simulink subsystem "Driving"  (R2024a)
settings: Solver=VariableStepAuto  StartTime=0.0  StopTime=10.0  RelTol=1e-3
settings Model: Creator=User  LastModifiedBy=User

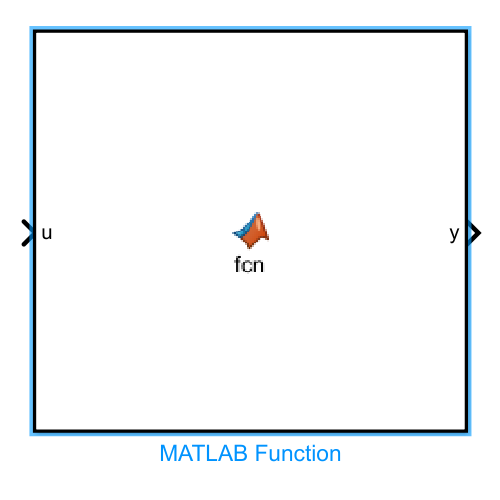
[thumbnail: Simulink's stored preview of the top-level diagram]
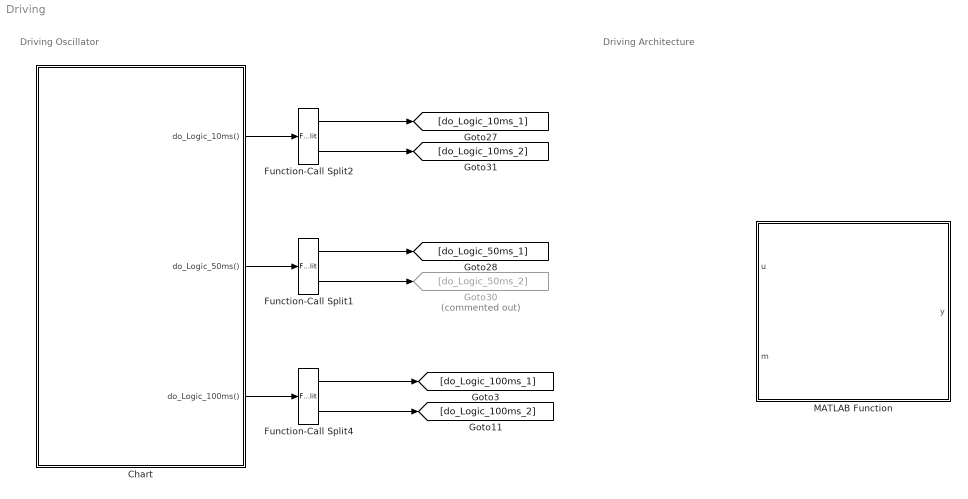
== system Driving ==
  note: Driving Oscillator
  note: Driving Architecture
  Chart : Stateflow chart  TreatAsAtomicUnit=on
  Function-Call Split1 : FunctionCallSplit  IconShape=distinctive  NumOutputPorts=2  OutputPortLayout=default
  Function-Call Split2 : FunctionCallSplit  IconShape=distinctive  NumOutputPorts=2  OutputPortLayout=default
  Function-Call Split4 : FunctionCallSplit  IconShape=distinctive  NumOutputPorts=2  OutputPortLayout=default
  Goto30 : Goto  Commented=on  GotoTag=do_Logic_50ms_2
  MATLAB Function : MATLAB Function  TreatAsAtomicUnit=on
  wires:
  Function-Call Split4/2 -> [do_Logic_100ms_2]
  Function-Call Split4/1 -> [do_Logic_100ms_1]
  Function-Call Split1/1 -> [do_Logic_50ms_1]
  Chart/3(do_Logic_100ms()) -> Function-Call Split4/1
  Function-Call Split2/2 -> [do_Logic_10ms_2]
  Function-Call Split1/2 -> Goto30/1
  Function-Call Split2/1 -> [do_Logic_10ms_1]
  Chart/2(do_Logic_50ms()) -> Function-Call Split1/1
  Chart/1(do_Logic_10ms()) -> Function-Call Split2/1

== matlab function Driving/MATLAB Function ==
  data: u input; y output; m input
function y = Driving(u, m)

y = u;

== stateflow chart Driving/Chart ==
  (default) -> (junction 1)
  (junction 1) -> (junction 3) [order 1] : [mod(i,10) == 0]
      | {do_Logic_10ms;}
  (junction 1) -> (junction 7) [order 2]
  (junction 3) -> (junction 5)
  (junction 5) -> (junction 7)
  (junction 7) -> (junction 10)
  (junction 10) -> (junction 12) [order 1] : [mod(i, 50) == 0]
      | {do_Logic_50ms;}
  (junction 10) -> (junction 18) [order 2]
  (junction 12) -> (junction 16)
  (junction 16) -> (junction 18)
  (junction 18) -> (junction 25)
  (junction 25) -> (junction 27) [order 1] : [mod(i,100) == 0]
      | {do_Logic_100ms;}
  (junction 25) -> (junction 21) [order 2]
  (junction 27) -> (junction 29) : {i = 0;}
  (junction 29) -> (junction 21)
  (junction 21) -> (junction 32) : {i = i +1;}
  data: i local =0
  events: do_Logic_10ms output FUNCTION_CALL_EVENT; do_Logic_50ms output FUNCTION_CALL_EVENT; do_Logic_100ms output FUNCTION_CALL_EVENT
